simulink model "DroopControl"  (R2025b)
settings: Solver=VariableStepAuto  StartTime=0.0  StopTime=0.3  MaxStep=1/20e3/100  RelTol=1e-3
InitFcn:
  | fs = 20000;
  | Ts = 1/fs;
  | I2B = 10;
  | UB = 20;
  | freq0 = 50;
  | freqc = 0.29999999999999999;
  | w0 = 2*pi*freq0;
  | wc = 2*pi*freqc;
  | I2_Kp = 3.023;
  | I2_Kr = 16.36;
  | Uc_Kp = 0.010579843316015665;
  | Uc_Kr = 0.56544574743993026;
  | I1_Kpi = 1.73;
  | UDC = 48;
  | Ic_Kd = 0;
  | Ts2 = 1/500;
  | 
  | %% 20V / 12A droop-grid configuration
  | % wc_grid is separate from the existing QPR parameter wc.
  | Grid_Condition = 'STRONG'; % STRONG / WEAK_INDUCTIVE / WEAK_RESISTIVE
  | fn = 50;
  | wn = 2*pi*fn;
  | E0 = 20; % phase-voltage peak, V
  | I_base = 12; % current peak, A
  | S_inv = 1.5*E0*I_base;
  | Z_base = E0/I_base;
  | switch Grid_Condition
  |     case 'STRONG'
  |         SCR = 10;
  |         XR_ratio = 5;
  |         Sn = 10*S_inv;
  |         delta_f_max = 0.2;
  |         delta_E_max = 0.02*E0;
  |         grid_wc = 25; % power-filter cutoff, rad/s
  |     case 'WEAK_INDUCTIVE'
  |         SCR = 1.5;
  |         XR_ratio = 3;
  |         Sn = 1.5*S_inv;
  |         delta_f_max = 1.5;
  |         delta_E_max = 0.10*E0;
  |         grid_wc = 120;
  |     case 'WEAK_RESISTIVE'
  |         SCR = 1.5;
  |         XR_ratio = 1;
  |         Sn = 1.5*S_inv;
  |         delta_f_max = 1.5;
  |         delta_E_max = 0.10*E0;
  |         grid_wc = 120;
  |     otherwise
  |         error('DroopGrid:InvalidCondition','Unknown Grid_Condition: %s',Grid_Condition);
  | end
  | Z_grid = Z_base/SCR;
  | Rg_val = Z_grid/sqrt(1+XR_ratio^2);
  | Lg_val = Rg_val*XR_ratio/wn;
  | grid_mp = 2*pi*delta_f_max/Sn;
  | grid_nq = delta_E_max/Sn;
  | grid_p0 = 0;
  | grid_q0 = 0;
  | Ts_ctrl = 1e-4; % actual droop-grid update period, 10 kHz
  | 
  | %% Physical-unit voltage/current cascade parameters (2026-10-03)
  | LCL_L1 = 200e-6;
  | LCL_L2 = 47e-6;
  | LCL_C = 1.8e-05;
  | LCL_R1 = 0.029999999999999999;
  | LCL_R2 = 0.014999999999999999;
  | I_meas_base = 1; % Clarke output in A, without current normalization
  | U_meas_base = 1; % Clarke output in V, without voltage normalization
  | PWM_Vbase = 1; % SVPWM input in V; conversion gain is unity
  | % Original QPR code has resonant gain 2*Kr at its center frequency.
  | % Imported Kr is interpreted using 2*Kr*wc*s/(s^2+2*wc*s+w0^2).
  | Uc_Kr_Code = Uc_Kr/2;
  | % Analysis metadata only; these do not add a delay/Pade block.
  | Design_delay_s = 5.4999999999999995e-05;
  | Design_pade_order = 2;
  | 
  | % Imported conservative controller profile (2026-10-04)
  | % Source export: 2026-10-04T06:14:23.773Z
  | % QPR fixed center 50 Hz; controller input latch and presync follow selected experiment.
  | % Design_delay_s is analysis metadata, not an additional runtime delay.
  | % Inverter-side loads are Resistor1/4/5; grid-side loads unchanged.
model workspace (MAT data in the model file):
  CurrentTestFinalPeak = 0.3
  CurrentTestInitialPeak = 0.1
  CurrentTestSignedStepTime = 0.03
libraries: nesl_utility x31, fl_lib x28, ee_lib x27, simulink x1, eePowerMeasurement x1
(part 1 of 2)
settings Model: Creator=GoodUser  LastModifiedBy=GoodUser

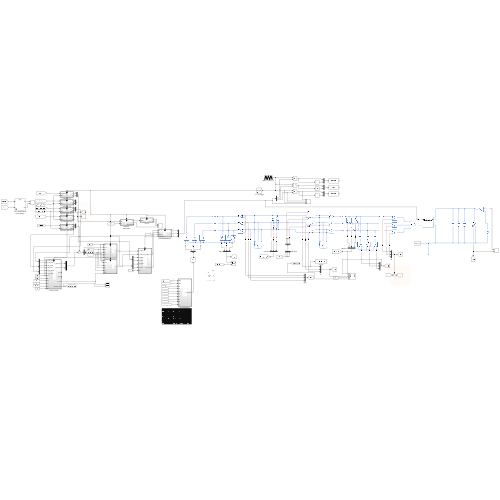
[thumbnail: Simulink's stored preview of the top-level diagram]
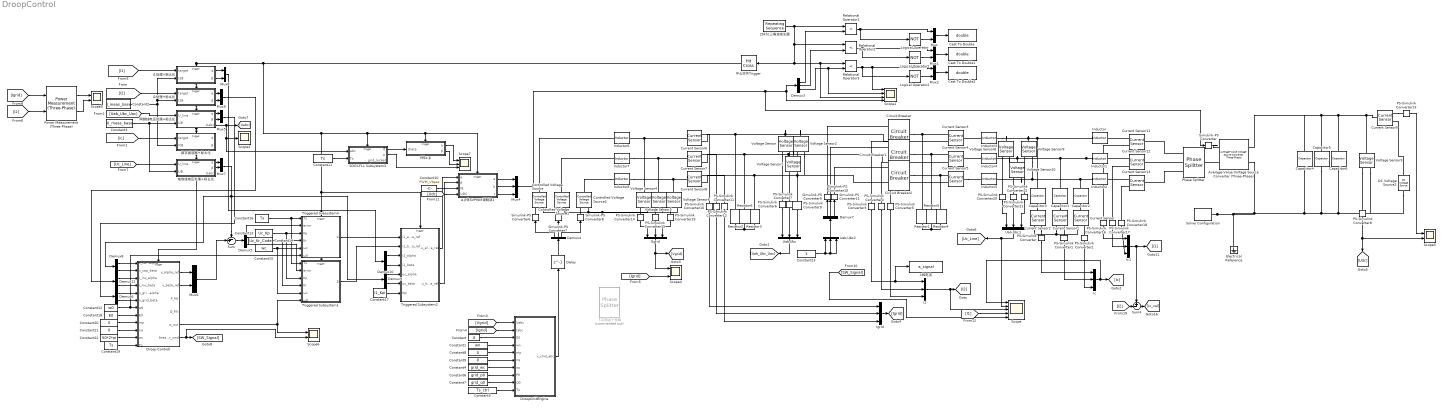
== system DroopControl ==
  20khz三角波发生器 : simulink/Sources/Repeating Sequence  rep_seq_t=[0 Ts/2 Ts]  rep_seq_y=[0 1 0]
  Average-Value Voltage Source Converter (Three-Phase) : ee_lib/Semiconductors & Converters/Converters/Average-Value Voltage Source Converter (Three-Phase)  port_option=ee.enum.threePhasePort.composite  frequency_option=ee.enum.converters.frequency.variable  input_option=ee.enum.converters.inputOption.ModWave  FRated=60 Hz  losses_parameterization=ee.enum.converters.losses.fixed  Pfixed=1 W  ks=0.01  kc1=1.7 V  kc2=0.01 Ohm  Ploss_vect=[100, 800, 1870, 3250, 4900] W  Irms_vect=[10, 100, 200, 300, 400] A  Vdc_nom=300 V  thermal_mass=30000 J/K  temperature_specify=off  temperature_priority=High  temperature=298.15 K  temperature_nominal_specify=off  temperature_nominal_value=1  temperature_nominal_unit=K
      settings: InternalSimscapePortConfiguration="{\"Bottom\":[],\"Left\":[{\"id\":\"ModWave\",\"label\":\"ModWave\",\"type\":\"input\"},{\"id\":\"N\",\"label\":\"~\",\"type\":\"foundation.electrical.three_phase\"}],\"Right\":[{\"id\":\"p\",\"label\":\"+\",\"type\":\"foundation.electrical.electrical\"},{\"id\":\"n\",\"label\":\"-\",\"type\":\"foundation.electrical.electrical\"}],\"Top\":[]}"
  A相电流 : ToWorkspace  VariableName=a_signal  SaveFormat=Timeseries  SampleTime=-1
  Capacitor1 : ee_lib/Passive/Capacitor  cap_option=ee.enum.passive.capacitor.capOption.const  c=LCL_C F  Cvec=[1e-05, 1e-06] F  Vvec=[0, 10] V  CV_table_symmetry=ee.enum.passive.capacitor.tableSymmetry.yes  f_vec=[1, 10] kHz  DFext_vec=[.8, 1.2]  enable_C_tol=ee.enum.toleranceApplication.none  averaging_period=0 s  C_tol=5  tol_distribution=ee.enum.toleranceDistribution.uniform  nSigma=4  r=8e-3 Ohm  g=0 1/Ohm  enable_operating_limits=ee.enum.enable.no  operating_limit_action=ee.enum.passive.reportOpLim.warn  max_working_voltage_range=[-25, 25] V  power_rating=1 W  maxTemperature=85 degC  thermalEnable=false  thermalMass=1 J/K  i_specify=off  i_priority=None  i=0 A  i_nominal_specify=off  i_nominal_value=1  i_nominal_unit=A  v_specify=off  v_priority=None  v=0 V  v_nominal_specify=off  v_nominal_value=1  v_nominal_unit=V  vc_specify=off  vc_priority=High  vc=0 V  vc_nominal_specify=off  vc_nominal_value=1  vc_nominal_unit=V  T_specify=off  T_priority=None  T=298.15 K  T_nominal_specify=off  T_nominal_value=1  T_nominal_unit=K
  Capacitor2 : ee_lib/Passive/Capacitor  cap_option=ee.enum.passive.capacitor.capOption.const  c=LCL_C F  Cvec=[1e-05, 1e-06] F  Vvec=[0, 10] V  CV_table_symmetry=ee.enum.passive.capacitor.tableSymmetry.yes  f_vec=[1, 10] kHz  DFext_vec=[.8, 1.2]  enable_C_tol=ee.enum.toleranceApplication.none  averaging_period=0 s  C_tol=5  tol_distribution=ee.enum.toleranceDistribution.uniform  nSigma=4  r=8e-3 Ohm  g=0 1/Ohm  enable_operating_limits=ee.enum.enable.no  operating_limit_action=ee.enum.passive.reportOpLim.warn  max_working_voltage_range=[-25, 25] V  power_rating=1 W  maxTemperature=85 degC  thermalEnable=false  thermalMass=1 J/K  i_specify=off  i_priority=None  i=0 A  i_nominal_specify=off  i_nominal_value=1  i_nominal_unit=A  v_specify=off  v_priority=None  v=0 V  v_nominal_specify=off  v_nominal_value=1  v_nominal_unit=V  vc_specify=off  vc_priority=High  vc=0 V  vc_nominal_specify=off  vc_nominal_value=1  vc_nominal_unit=V  T_specify=off  T_priority=None  T=298.15 K  T_nominal_specify=off  T_nominal_value=1  T_nominal_unit=K
  Capacitor3 : ee_lib/Passive/Capacitor  cap_option=ee.enum.passive.capacitor.capOption.const  c=LCL_C F  Cvec=[1e-05, 1e-06] F  Vvec=[0, 10] V  CV_table_symmetry=ee.enum.passive.capacitor.tableSymmetry.yes  f_vec=[1, 10] kHz  DFext_vec=[.8, 1.2]  enable_C_tol=ee.enum.toleranceApplication.none  averaging_period=0 s  C_tol=5  tol_distribution=ee.enum.toleranceDistribution.uniform  nSigma=4  r=8e-3 Ohm  g=0 1/Ohm  enable_operating_limits=ee.enum.enable.no  operating_limit_action=ee.enum.passive.reportOpLim.warn  max_working_voltage_range=[-25, 25] V  power_rating=1 W  maxTemperature=85 degC  thermalEnable=false  thermalMass=1 J/K  i_specify=off  i_priority=None  i=0 A  i_nominal_specify=off  i_nominal_value=1  i_nominal_unit=A  v_specify=off  v_priority=None  v=0 V  v_nominal_specify=off  v_nominal_value=1  v_nominal_unit=V  vc_specify=off  vc_priority=High  vc=0 V  vc_nominal_specify=off  vc_nominal_value=1  vc_nominal_unit=V  T_specify=off  T_priority=None  T=298.15 K  T_nominal_specify=off  T_nominal_value=1  T_nominal_unit=K
  Capacitor4 : ee_lib/Passive/Capacitor  cap_option=ee.enum.passive.capacitor.capOption.const  c=0.001 F  Cvec=[1e-05, 1e-06] F  Vvec=[0, 10] V  CV_table_symmetry=ee.enum.passive.capacitor.tableSymmetry.yes  f_vec=[1, 10] kHz  DFext_vec=[.8, 1.2]  enable_C_tol=ee.enum.toleranceApplication.none  averaging_period=0 s  C_tol=5  tol_distribution=ee.enum.toleranceDistribution.uniform  nSigma=4  r=200e-3 Ohm  g=0 1/Ohm  enable_operating_limits=ee.enum.enable.no  operating_limit_action=ee.enum.passive.reportOpLim.warn  max_working_voltage_range=[-25, 25] V  power_rating=1 W  maxTemperature=85 degC  thermalEnable=false  thermalMass=1 J/K  i_specify=off  i_priority=None  i=0 A  i_nominal_specify=off  i_nominal_value=1  i_nominal_unit=A  v_specify=on  v_priority=None  v=34.641 V  v_nominal_specify=off  v_nominal_value=1  v_nominal_unit=V  vc_specify=on  vc_priority=High  vc=34.641 V  vc_nominal_specify=off  vc_nominal_value=1  vc_nominal_unit=V  T_specify=off  T_priority=None  T=298.15 K  T_nominal_specify=off  T_nominal_value=1  T_nominal_unit=K
  Capacitor5 : ee_lib/Passive/Capacitor  cap_option=ee.enum.passive.capacitor.capOption.const  c=0.001 F  Cvec=[1e-05, 1e-06] F  Vvec=[0, 10] V  CV_table_symmetry=ee.enum.passive.capacitor.tableSymmetry.yes  f_vec=[1, 10] kHz  DFext_vec=[.8, 1.2]  enable_C_tol=ee.enum.toleranceApplication.none  averaging_period=0 s  C_tol=5  tol_distribution=ee.enum.toleranceDistribution.uniform  nSigma=4  r=200e-3 Ohm  g=0 1/Ohm  enable_operating_limits=ee.enum.enable.no  operating_limit_action=ee.enum.passive.reportOpLim.warn  max_working_voltage_range=[-25, 25] V  power_rating=1 W  maxTemperature=85 degC  thermalEnable=false  thermalMass=1 J/K  i_specify=off  i_priority=None  i=0 A  i_nominal_specify=off  i_nominal_value=1  i_nominal_unit=A  v_specify=on  v_priority=None  v=34.641 V  v_nominal_specify=off  v_nominal_value=1  v_nominal_unit=V  vc_specify=on  vc_priority=High  vc=34.641 V  vc_nominal_specify=off  vc_nominal_value=1  vc_nominal_unit=V  T_specify=off  T_priority=None  T=298.15 K  T_nominal_specify=off  T_nominal_value=1  T_nominal_unit=K
  Capacitor6 : ee_lib/Passive/Capacitor  cap_option=ee.enum.passive.capacitor.capOption.const  c=0.001 F  Cvec=[1e-05, 1e-06] F  Vvec=[0, 10] V  CV_table_symmetry=ee.enum.passive.capacitor.tableSymmetry.yes  f_vec=[1, 10] kHz  DFext_vec=[.8, 1.2]  enable_C_tol=ee.enum.toleranceApplication.none  averaging_period=0 s  C_tol=5  tol_distribution=ee.enum.toleranceDistribution.uniform  nSigma=4  r=200e-3 Ohm  g=0 1/Ohm  enable_operating_limits=ee.enum.enable.no  operating_limit_action=ee.enum.passive.reportOpLim.warn  max_working_voltage_range=[-25, 25] V  power_rating=1 W  maxTemperature=85 degC  thermalEnable=false  thermalMass=1 J/K  i_specify=off  i_priority=None  i=0 A  i_nominal_specify=off  i_nominal_value=1  i_nominal_unit=A  v_specify=on  v_priority=None  v=34.641 V  v_nominal_specify=off  v_nominal_value=1  v_nominal_unit=V  vc_specify=on  vc_priority=High  vc=34.641 V  vc_nominal_specify=off  vc_nominal_value=1  vc_nominal_unit=V  T_specify=off  T_priority=None  T=298.15 K  T_nominal_specify=off  T_nominal_value=1  T_nominal_unit=K
  Cast To Double : DataTypeConversion  OutDataTypeStr=double  SaturateOnIntegerOverflow=off  RndMeth=Floor
  Cast To Double1 : DataTypeConversion  OutDataTypeStr=double  SaturateOnIntegerOverflow=off  RndMeth=Floor
  Cast To Double2 : DataTypeConversion  OutDataTypeStr=double  SaturateOnIntegerOverflow=off  RndMeth=Floor
  Circuit Breaker : ee_lib/Switches & Breakers/Circuit Breaker  R_closed=0.001 Ohm  G_open=1e-6 1/Ohm  threshold=0.5 V  breaker_behavior=ee.enum.switches.breakerBehavior.zeroCrossingEnable
      settings: InternalSimscapePortConfiguration="{\"Bottom\":[],\"Left\":[{\"id\":\"vT\",\"label\":\"vT\",\"type\":\"input\"},{\"id\":\"p1\",\"label\":\"\",\"type\":\"foundation.electrical.electrical\"}],\"Right\":[{\"id\":\"p2\",\"label\":\"\",\"type\":\"foundation.electrical.electrical\"}],\"Top\":[]}"
  Circuit Breaker1 : ee_lib/Switches & Breakers/Circuit Breaker  R_closed=0.001 Ohm  G_open=1e-6 1/Ohm  threshold=0.5 V  breaker_behavior=ee.enum.switches.breakerBehavior.zeroCrossingEnable
      settings: InternalSimscapePortConfiguration="{\"Bottom\":[],\"Left\":[{\"id\":\"vT\",\"label\":\"vT\",\"type\":\"input\"},{\"id\":\"p1\",\"label\":\"\",\"type\":\"foundation.electrical.electrical\"}],\"Right\":[{\"id\":\"p2\",\"label\":\"\",\"type\":\"foundation.electrical.electrical\"}],\"Top\":[]}"
  Circuit Breaker2 : ee_lib/Switches & Breakers/Circuit Breaker  R_closed=0.001 Ohm  G_open=1e-6 1/Ohm  threshold=1 V  breaker_behavior=ee.enum.switches.breakerBehavior.zeroCrossingEnable
      settings: InternalSimscapePortConfiguration="{\"Bottom\":[],\"Left\":[{\"id\":\"vT\",\"label\":\"vT\",\"type\":\"input\"},{\"id\":\"p1\",\"label\":\"\",\"type\":\"foundation.electrical.electrical\"}],\"Right\":[{\"id\":\"p2\",\"label\":\"\",\"type\":\"foundation.electrical.electrical\"}],\"Top\":[]}"
  Constant{,8..9,20..21} (5 alike) : Constant  Value=0
  Constant1 : Constant  Value=wn
  Constant10 : Constant  Value=PWM_Vbase
  Constant11 : Constant  Value=Ts
  Constant12 : Constant  Value=w0
  Constant13 : Constant  Value=Uc_Kp
  Constant14 : Constant  Value=Uc_Kr_Code
  Constant15 : Constant  Value=wc
  Constant16 : Constant  Value=Ts
  Constant17 : Constant  Value=I1_Kpi
  Constant18 : Constant  Value=E0
  Constant19 : Constant  Value=Ts
  Constant2 : Constant  Value=I_meas_base
  Constant22 : Constant  Value=50*2*pi
  Constant23 : Constant
  Constant3 : Constant  Value=U_meas_base
  Constant4 : Constant  Value=grid_wc
  Constant5 : Constant  Value=Ts_ctrl
  Constant6 : Constant  Value=grid_p0
  Constant7 : Constant  Value=grid_q0
  Controlled Voltage Source : fl_lib/Electrical/Electrical Sources/Controlled Voltage Source
  Controlled Voltage Source1 : fl_lib/Electrical/Electrical Sources/Controlled Voltage Source
  Controlled Voltage Source2 : fl_lib/Electrical/Electrical Sources/Controlled Voltage Source
  Current Sensor{,1..9,11..13} (13 alike) : fl_lib/Electrical/Electrical Sensors/Current Sensor
  DC Voltage Source2 : fl_lib/Electrical/Electrical Sources/DC Voltage Source  v0=48 V
  Delay : Delay  DelayLength=1  InitialCondition=0
  Demux{5..6,8..11} (6 alike) : Demux  Outputs=2
  Demux3 : Demux  Outputs=3
  Demux4 : Demux  Outputs=3
  Demux7 : Demux  Outputs=3
  "Droop Controll " : Subsystem  TreatAsAtomicUnit=on
  DroopGridEngine : Subsystem  TreatAsAtomicUnit=on
  Electrical Reference : fl_lib/Electrical/Electrical Elements/Electrical Reference
  Ggrid : Mux  Inputs=3
  I1处理+标幺化 : Subsystem  TreatAsAtomicUnit=on
  I2 : Mux  Inputs=3
  I2处理+标幺化 : Subsystem  TreatAsAtomicUnit=on
  Ic : Mux  Inputs=3
  Ic1 : Mux  Inputs=3
  Igrid : Mux  Inputs=3
  Inductor : ee_lib/Passive/Inductor  l=LCL_L1 H  enable_L_tol=ee.enum.toleranceApplication.none  L_tol=20  tol_distribution=ee.enum.toleranceDistribution.uniform  nSigma=4  r=LCL_R1 Ohm  g=1e-9 1/Ohm  enable_operating_limits=ee.enum.enable.no  operating_limit_action=ee.enum.passive.reportOpLim.warn  max_working_current=1 A  power_rating=1 W  i_L_specify=off  i_L_priority=High  i_L=0 A  i_L_nominal_specify=off  i_L_nominal_value=1  i_L_nominal_unit=A
  Inductor1 : ee_lib/Passive/Inductor  l=LCL_L1 H  enable_L_tol=ee.enum.toleranceApplication.none  L_tol=20  tol_distribution=ee.enum.toleranceDistribution.uniform  nSigma=4  r=LCL_R1 Ohm  g=1e-9 1/Ohm  enable_operating_limits=ee.enum.enable.no  operating_limit_action=ee.enum.passive.reportOpLim.warn  max_working_current=1 A  power_rating=1 W  i_L_specify=off  i_L_priority=High  i_L=0 A  i_L_nominal_specify=off  i_L_nominal_value=1  i_L_nominal_unit=A
  Inductor2 : ee_lib/Passive/Inductor  l=LCL_L1 H  enable_L_tol=ee.enum.toleranceApplication.none  L_tol=20  tol_distribution=ee.enum.toleranceDistribution.uniform  nSigma=4  r=LCL_R1 Ohm  g=1e-9 1/Ohm  enable_operating_limits=ee.enum.enable.no  operating_limit_action=ee.enum.passive.reportOpLim.warn  max_working_current=1 A  power_rating=1 W  i_L_specify=off  i_L_priority=High  i_L=0 A  i_L_nominal_specify=off  i_L_nominal_value=1  i_L_nominal_unit=A
  Inductor3 : ee_lib/Passive/Inductor  l=LCL_L2 H  enable_L_tol=ee.enum.toleranceApplication.none  L_tol=20  tol_distribution=ee.enum.toleranceDistribution.uniform  nSigma=4  r=LCL_R2 Ohm  g=1e-9 1/Ohm  enable_operating_limits=ee.enum.enable.no  operating_limit_action=ee.enum.passive.reportOpLim.warn  max_working_current=1 A  power_rating=1 W  i_L_specify=off  i_L_priority=High  i_L=0 A  i_L_nominal_specify=off  i_L_nominal_value=1  i_L_nominal_unit=A
  Inductor4 : ee_lib/Passive/Inductor  l=LCL_L2 H  enable_L_tol=ee.enum.toleranceApplication.none  L_tol=20  tol_distribution=ee.enum.toleranceDistribution.uniform  nSigma=4  r=LCL_R2 Ohm  g=1e-9 1/Ohm  enable_operating_limits=ee.enum.enable.no  operating_limit_action=ee.enum.passive.reportOpLim.warn  max_working_current=1 A  power_rating=1 W  i_L_specify=off  i_L_priority=High  i_L=0 A  i_L_nominal_specify=off  i_L_nominal_value=1  i_L_nominal_unit=A
  Inductor5 : ee_lib/Passive/Inductor  l=LCL_L2 H  enable_L_tol=ee.enum.toleranceApplication.none  L_tol=20  tol_distribution=ee.enum.toleranceDistribution.uniform  nSigma=4  r=LCL_R2 Ohm  g=1e-9 1/Ohm  enable_operating_limits=ee.enum.enable.no  operating_limit_action=ee.enum.passive.reportOpLim.warn  max_working_current=1 A  power_rating=1 W  i_L_specify=off  i_L_priority=High  i_L=0 A  i_L_nominal_specify=off  i_L_nominal_value=1  i_L_nominal_unit=A
  Inductor6 : ee_lib/Passive/Inductor  l=Lg_val H  enable_L_tol=ee.enum.toleranceApplication.none  L_tol=20  tol_distribution=ee.enum.toleranceDistribution.uniform  nSigma=4  r=Rg_val Ohm  g=1e-9 1/Ohm  enable_operating_limits=ee.enum.enable.no  operating_limit_action=ee.enum.passive.reportOpLim.warn  max_working_current=1 A  power_rating=1 W  i_L_specify=off  i_L_priority=High  i_L=0 A  i_L_nominal_specify=off  i_L_nominal_value=1  i_L_nominal_unit=A
  Inductor7 : ee_lib/Passive/Inductor  l=Lg_val H  enable_L_tol=ee.enum.toleranceApplication.none  L_tol=20  tol_distribution=ee.enum.toleranceDistribution.uniform  nSigma=4  r=Rg_val Ohm  g=1e-9 1/Ohm  enable_operating_limits=ee.enum.enable.no  operating_limit_action=ee.enum.passive.reportOpLim.warn  max_working_current=1 A  power_rating=1 W  i_L_specify=off  i_L_priority=High  i_L=0 A  i_L_nominal_specify=off  i_L_nominal_value=1  i_L_nominal_unit=A
  Inductor8 : ee_lib/Passive/Inductor  l=Lg_val H  enable_L_tol=ee.enum.toleranceApplication.none  L_tol=20  tol_distribution=ee.enum.toleranceDistribution.uniform  nSigma=4  r=Rg_val Ohm  g=1e-9 1/Ohm  enable_operating_limits=ee.enum.enable.no  operating_limit_action=ee.enum.passive.reportOpLim.warn  max_working_current=1 A  power_rating=1 W  i_L_specify=off  i_L_priority=High  i_L=0 A  i_L_nominal_specify=off  i_L_nominal_value=1  i_L_nominal_unit=A
  Logical Operator : Logic  Operator=NOT  AllPortsSameDT=off  OutDataTypeStr=boolean
  Logical Operator1 : Logic  Operator=NOT  AllPortsSameDT=off  OutDataTypeStr=boolean
  Logical Operator2 : Logic  Operator=NOT  AllPortsSameDT=off  OutDataTypeStr=boolean
  Mux{,1..2,5..9} (8 alike) : Mux  Inputs=2
  Mux4 : Mux  Inputs=3
  PS-Simulink Converter{,1..22} (23 alike) : nesl_utility/PS-Simulink Converter  PhysicalDomain=network_engine_domain  SubClassName=ps_output  LeftPortType=input  RightPortType=output  PseudoPeriodic=off  Frequencies=[]  VectorFormat=inherit  Unit=inherit  AffineConversion=off
  Phase Splitter : ee_lib/Connectors & References/Phase Splitter
  Power Measurement (Three-Phase) : eePowerMeasurement/Power Measurement (Three-Phase)  LabelModeActiveChoice=Continuous  F=60  K=[0 1 2 3]  Seq=Positive  Ts=0
  Relational Operator1 : RelationalOperator  Operator=<  OutDataTypeStr=boolean  RndMeth=Simplest  InputSameDT=off
  Relational Operator2 : RelationalOperator  Operator=<  OutDataTypeStr=boolean  RndMeth=Simplest  InputSameDT=off
  Relational Operator3 : RelationalOperator  Operator=<  OutDataTypeStr=boolean  RndMeth=Simplest  InputSameDT=off
  Resistor1 : ee_lib/Passive/Resistor  R=50 Ohm  enable_R_tol=ee.enum.toleranceApplication.none  R_tol=5  tol_distribution=ee.enum.toleranceDistribution.uniform  nSigma=4  enable_operating_limits=ee.enum.enable.no  operating_limit_action=ee.enum.passive.reportOpLim.warn  power_rating=1 W  max_working_voltage=100 V  noise_mode=ee.enum.sources.noise.Disabled  Tdevice=25 degC  sample_time=1e-3 s  repeatability=ee.enum.ic.repeatability.notRepeatable  user_seed=0  auto_seed=3499211588  power_derating_T1=70 degC  power_derating_T2=155 degC  operating_temperature_range_vec=[-50, 150] degC  alpha=3.93e-3 1/K  Tmeas=25 degC  thermal_mass=100 J/K  temperature_specify=off  temperature_priority=High  temperature=298.15 K  temperature_nominal_specify=off  temperature_nominal_value=1  temperature_nominal_unit=K
  Resistor2 : ee_lib/Passive/Resistor  R=100 Ohm  enable_R_tol=ee.enum.toleranceApplication.none  R_tol=5  tol_distribution=ee.enum.toleranceDistribution.uniform  nSigma=4  enable_operating_limits=ee.enum.enable.no  operating_limit_action=ee.enum.passive.reportOpLim.warn  power_rating=1 W  max_working_voltage=100 V  noise_mode=ee.enum.sources.noise.Disabled  Tdevice=25 degC  sample_time=1e-3 s  repeatability=ee.enum.ic.repeatability.notRepeatable  user_seed=0  auto_seed=1826474873  power_derating_T1=70 degC  power_derating_T2=155 degC  operating_temperature_range_vec=[-50, 150] degC  alpha=3.93e-3 1/K  Tmeas=25 degC  thermal_mass=100 J/K  temperature_specify=off  temperature_priority=High  temperature=298.15 K  temperature_nominal_specify=off  temperature_nominal_value=1  temperature_nominal_unit=K
  Resistor3 : ee_lib/Passive/Resistor  R=100 Ohm  enable_R_tol=ee.enum.toleranceApplication.none  R_tol=5  tol_distribution=ee.enum.toleranceDistribution.uniform  nSigma=4  enable_operating_limits=ee.enum.enable.no  operating_limit_action=ee.enum.passive.reportOpLim.warn  power_rating=1 W  max_working_voltage=100 V  noise_mode=ee.enum.sources.noise.Disabled  Tdevice=25 degC  sample_time=1e-3 s  repeatability=ee.enum.ic.repeatability.notRepeatable  user_seed=0  auto_seed=693571696  power_derating_T1=70 degC  power_derating_T2=155 degC  operating_temperature_range_vec=[-50, 150] degC  alpha=3.93e-3 1/K  Tmeas=25 degC  thermal_mass=100 J/K  temperature_specify=off  temperature_priority=High  temperature=298.15 K  temperature_nominal_specify=off  temperature_nominal_value=1  temperature_nominal_unit=K
  Resistor4 : ee_lib/Passive/Resistor  R=50 Ohm  enable_R_tol=ee.enum.toleranceApplication.none  R_tol=5  tol_distribution=ee.enum.toleranceDistribution.uniform  nSigma=4  enable_operating_limits=ee.enum.enable.no  operating_limit_action=ee.enum.passive.reportOpLim.warn  power_rating=1 W  max_working_voltage=100 V  noise_mode=ee.enum.sources.noise.Disabled  Tdevice=25 degC  sample_time=1e-3 s  repeatability=ee.enum.ic.repeatability.notRepeatable  user_seed=0  auto_seed=3890346746  power_derating_T1=70 degC  power_derating_T2=155 degC  operating_temperature_range_vec=[-50, 150] degC  alpha=3.93e-3 1/K  Tmeas=25 degC  thermal_mass=100 J/K  temperature_specify=off  temperature_priority=High  temperature=298.15 K  temperature_nominal_specify=off  temperature_nominal_value=1  temperature_nominal_unit=K
  Resistor5 : ee_lib/Passive/Resistor  R=50 Ohm  enable_R_tol=ee.enum.toleranceApplication.none  R_tol=5  tol_distribution=ee.enum.toleranceDistribution.uniform  nSigma=4  enable_operating_limits=ee.enum.enable.no  operating_limit_action=ee.enum.passive.reportOpLim.warn  power_rating=1 W  max_working_voltage=100 V  noise_mode=ee.enum.sources.noise.Disabled  Tdevice=25 degC  sample_time=1e-3 s  repeatability=ee.enum.ic.repeatability.notRepeatable  user_seed=0  auto_seed=545404223  power_derating_T1=70 degC  power_derating_T2=155 degC  operating_temperature_range_vec=[-50, 150] degC  alpha=3.93e-3 1/K  Tmeas=25 degC  thermal_mass=100 J/K  temperature_specify=off  temperature_priority=High  temperature=298.15 K  temperature_nominal_specify=off  temperature_nominal_value=1  temperature_nominal_unit=K
  Resistor6 : ee_lib/Passive/Resistor  R=100 Ohm  enable_R_tol=ee.enum.toleranceApplication.none  R_tol=5  tol_distribution=ee.enum.toleranceDistribution.uniform  nSigma=4  enable_operating_limits=ee.enum.enable.no  operating_limit_action=ee.enum.passive.reportOpLim.warn  power_rating=1 W  max_working_voltage=100 V  noise_mode=ee.enum.sources.noise.Disabled  Tdevice=25 degC  sample_time=1e-3 s  repeatability=ee.enum.ic.repeatability.notRepeatable  user_seed=0  auto_seed=1343117392  power_derating_T1=70 degC  power_derating_T2=155 degC  operating_temperature_range_vec=[-50, 150] degC  alpha=3.93e-3 1/K  Tmeas=25 degC  thermal_mass=100 J/K  temperature_specify=off  temperature_priority=High  temperature=298.15 K  temperature_nominal_specify=off  temperature_nominal_value=1  temperature_nominal_unit=K
  SOGI-FLL Subsystem3 : Subsystem  TreatAsAtomicUnit=on
  Scope : Scope  NumInputPorts=5
      settings: ActiveDisplayYMinimum=-0.75702904285827766  ActiveDisplayYMaximum=0.7141001708324739
  Scope1 : Scope  NumInputPorts=4
      settings: ActiveDisplayYMinimum=-0.2219648833427319  ActiveDisplayYMaximum=1.3978468617731235
  Scope2 : Scope
      settings: ActiveDisplayYMinimum=-3.6838007228839231  ActiveDisplayYMaximum=2.775125553261212  DataLoggingVariableName=ScopeData2
  Scope{3..6} (4 alike) : Scope  NumInputPorts=2
      Scope3 settings: ActiveDisplayYMinimum=-5.9984838768546282  ActiveDisplayYMaximum=54.67249551752824  DataLoggingVariableName=ScopeData3
      Scope4 settings: ActiveDisplayYMinimum=-26.098635713677506  ActiveDisplayYMaximum=27.193712323408977  DataLoggingVariableName=ScopeData4
      Scope5 settings: ActiveDisplayYMinimum=-940.793349498487  ActiveDisplayYMaximum=150.37889545432691  DataLoggingVariableName=ScopeData5
      Scope6 settings: ActiveDisplayYMinimum=-39.269908169872409  ActiveDisplayYMaximum=353.42917352885172  DataLoggingVariableName=ScopeData6
  Scope7 : Scope  NumInputPorts=3
      settings: ActiveDisplayYMinimum=287.341337897508  ActiveDisplayYMaximum=314.82598204167613  DataLoggingVariableName=ScopeData7
  Simulink-PS Converter{,6..11} (7 alike) : nesl_utility/Simulink-PS Converter  PhysicalDomain=network_engine_domain  SubClassName=ps_input  LeftPortType=input  RightPortType=output  PseudoPeriodic=off  Frequencies=[]  NoiseDistribution=none  NoiseParameters=[]  Unit=1  AffineConversion=off  FilteringAndDerivatives=provide  SimscapeFilterOrder=1  InputFilterTimeConstant=0.001  UdotUserProvided=0
  Solver Configuration : nesl_utility/Solver Configuration  PhysicalDomain=network_engine_domain  SubClassName=solver  LeftPortType=input  RightPortType=generic  Tones=[]  Harmonics=[]  SimulateNoise=off  Profile=off  UseLocalSampling=off  EnableSwitchedLinearOptims=on  FrequencyDomain=off  UseCCode=off  RelTol=0.001  AbsTol=0.001  MinStep=1e-09  ToWorkspace=off  RevertToSquareIcSolve=off  NumHomotopyIterations=100  PhasorMode=off  PhasorModeNumHarmonics=1  ConsistencySolver=NEWTON_XTOL_AFTER_FTOL  IndexReductionMethod=DerivativeReplacement  DoDC=off  ResidualTolerance=1e-09  ConsistencyTolSource=GLOBAL  ConsistencyAbsTol=0.001  ConsistencyRelTol=0.001  ConsistencyTolFactor=0.001  UseLocalSolver=on  LocalSolverChoice=NE_BACKWARD_EULER_ADVANCER  ResolveIndetEquations=on  FunctionEvalNumThread=1  LocalSolverSampleTime=1/20e3/100  DoFixedCost=off  MaxNonlinIter=3  MaxModeIter=2  ComputeImpulses=off  ImpulseIterations=2  LinearAlgebra=auto  LinearAlgebraNumThread=0  EquationFormulation=NE_TIME_EF  DelaysMemoryBudget=1024  AutomaticFiltering=on  FilteringTimeConstant=0.001  PartitionStorageMethod=AS_NEEDED  PartitionMemoryBudget=1024  PartitionMethod=ROBUST  MultibodyUseLocalSolver=off  MultibodyLocalSolverChoice=ODE1  MultibodyLocalSolverSampleTime=0.001
  Sum : Sum  Inputs=-+|
  Sum4 : Sum  Inputs=+-|
  Triggered Subsystem1 : Subsystem  TreatAsAtomicUnit=on
  Triggered Subsystem2 : Subsystem  TreatAsAtomicUnit=on
  Triggered Subsystem4 : Subsystem  TreatAsAtomicUnit=on
  Uab,Ubc : Mux  Inputs=3
  Uab,Ubc1 : Mux  Inputs=3
  Uab,Ubc2 : Mux  Inputs=3
  Voltage Sensor{,1..6,8..10} (10 alike) : fl_lib/Electrical/Electrical Sensors/Voltage Sensor
  α,β转SVPWM调制波1 : Subsystem  TreatAsAtomicUnit=on
  θ转α,β : Subsystem  TreatAsAtomicUnit=on
  下次用这个布线 : ee_lib/Connectors & References/Phase Splitter  Commented=on
  中心对齐Trigger : HitCross  HitCrossingOffset=0.00  HitCrossingDirection=rising
  数字滤波器+标幺化 : Subsystem  TreatAsAtomicUnit=on
  电容线电压处理+标幺化 : Subsystem  TreatAsAtomicUnit=on
  网侧线电压处理+标幺化 : Subsystem  TreatAsAtomicUnit=on
  wires:
  PS-Simulink Converter/1 -> Ic/1
  PS-Simulink Converter1/1 -> Ic/2
  PS-Simulink Converter2/1 -> Ic/3
  PS-Simulink Converter3/1 -> A相电流/1, I2/1
  PS-Simulink Converter4/1 -> I2/2
  PS-Simulink Converter5/1 -> I2/3
  PS-Simulink Converter7/1 -> Uab,Ubc/2
  PS-Simulink Converter6/1 -> Uab,Ubc/1
  Demux3/1 -> Relational Operator1/2
  Relational Operator2/1 -> Mux1/1, Logical Operator1/1
  Demux3/2 -> Relational Operator2/2
  20khz三角波发生器/1 -> Relational Operator1/1, 中心对齐Trigger/1, Scope1/3, Relational Operator3/1, Relational Operator2/1
  Demux3/3 -> Scope1/2, Relational Operator3/2
  Mux/1 -> Cast To Double/1
  Mux1/1 -> Cast To Double1/1
  Ic/1 -> Scope/1, [Ic]
  Logical Operator1/1 -> Mux1/2
  Logical Operator/1 -> Mux/2
  Logical Operator2/1 -> Mux2/2
  Mux2/1 -> Cast To Double2/1
  Relational Operator3/1 -> Logical Operator2/1, Scope1/1, Mux2/1
  Relational Operator1/1 -> Logical Operator/1, Mux/1
  中心对齐Trigger/1 -> I1处理+标幺化/Trigger, 网侧线电压处理+标幺化/Trigger, "Droop Controll "/Trigger, 电容线电压处理+标幺化/Trigger, 数字滤波器+标幺化/Trigger, I2处理+标幺化/Trigger, SOGI-FLL Subsystem3/Trigger, α,β转SVPWM调制波1/Trigger, θ转α,β/Trigger, Triggered Subsystem2/Trigger, Triggered Subsystem1/Trigger, Triggered Subsystem4/Trigger
  I2/1 -> Scope/3, [I2]
  Uab,Ubc/1 -> [Uab_Ubc_Uac]
  [I2] -> I2处理+标幺化/1(target)
  [Uab_Ubc_Uac] -> 网侧线电压处理+标幺化/1(U_line)
  网侧线电压处理+标幺化/3(Uabc) -> Scope2/1, SOGI-FLL Subsystem3/1(abc), [Uabc]
  PS-Simulink Converter9/1 -> Uab,Ubc/3
  Constant2/1 -> 数字滤波器+标幺化/2(ICB), I1处理+标幺化/2(I2B), I2处理+标幺化/2(I2B)
  Constant3/1 -> 电容线电压处理+标幺化/2(UB), 网侧线电压处理+标幺化/2(UB)
  SOGI-FLL Subsystem3/1(θ) -> θ转α,β/1(theta)
  [Ic] -> 数字滤波器+标幺化/1(target)
  PS-Simulink Converter8/1 -> Scope3/2, [Udc]
  PS-Simulink Converter10/1 -> Igrid/1
  PS-Simulink Converter11/1 -> Igrid/2
  PS-Simulink Converter12/1 -> Igrid/3
  PS-Simulink Converter13/1 -> Scope3/1
  [I2] -> Power Measurement (Three-Phase)/2
  [Igrid] -> Power Measurement (Three-Phase)/1
  Power Measurement (Three-Phase)/1 -> Scope5/1
  Power Measurement (Three-Phase)/2 -> Scope5/2
  PS-Simulink Converter16/1 -> Ic1/1
  PS-Simulink Converter17/1 -> Ic1/2
  PS-Simulink Converter18/1 -> Ic1/3
  Ic1/1 -> [I1], Sum4/1
  [I2] -> Sum4/2
  Sum4/1 -> [Ic_cal]
  Igrid/1 -> [Igrid]
  [I1] -> I1处理+标幺化/1(target)
  DroopGridEngine/1(v_cmd_abc) -> Delay/1
  Demux4/1 -> Simulink-PS Converter6/1
  Demux4/2 -> Simulink-PS Converter7/1
  Demux4/3 -> Simulink-PS Converter8/1
  PS-Simulink Converter14/1 -> Ggrid/1
  PS-Simulink Converter15/1 -> Ggrid/2
  PS-Simulink Converter19/1 -> Ggrid/3
  Ggrid/1 -> [Vgrid], Scope4/1
  [Igrid] -> DroopGridEngine/2(Iabc)
  [Vgrid] -> DroopGridEngine/1(Vabc)
  Constant/1 -> DroopGridEngine/3(E0)
  Constant1/1 -> DroopGridEngine/4(wn)
  Constant4/1 -> DroopGridEngine/7(wc)
  Constant5/1 -> DroopGridEngine/10(Ts)
  Constant7/1 -> DroopGridEngine/9(Q0)
  Constant6/1 -> DroopGridEngine/8(P0)
  Constant9/1 -> DroopGridEngine/6(nq)
  Constant8/1 -> DroopGridEngine/5(mp)
  Mux4/1 -> Simulink-PS Converter/1, Demux3/1, Scope1/4
  Delay/1 -> Demux4/1
  [Igrid] -> Scope4/2
  "Droop Controll "/1(v_alpha_ref) -> Mux6/1
  "Droop Controll "/2(v_beta_ref) -> Mux6/2
  Mux6/1 -> Sum/2
  Sum/1 -> Demux5/1
  Demux5/1 -> Triggered Subsystem4/2(error)
  Demux5/2 -> Triggered Subsystem1/2(error)
  PS-Simulink Converter20/1 -> Uab,Ubc1/1
  PS-Simulink Converter21/1 -> Uab,Ubc1/2
  PS-Simulink Converter22/1 -> Uab,Ubc1/3
  Uab,Ubc1/1 -> Scope/2, [Uc_Line]
  [Uc_Line] -> 电容线电压处理+标幺化/1(U_line)
  Mux5/1 -> Demux6/1
  网侧线电压处理+标幺化/1(α) -> Mux5/1
  网侧线电压处理+标幺化/2(β) -> Mux5/2
  Constant11/1 -> SOGI-FLL Subsystem3/2(Ts)
  Demux7/1 -> Simulink-PS Converter9/1
  Demux7/2 -> Simulink-PS Converter10/1
  Demux7/3 -> Simulink-PS Converter11/1
  [SW_Signal] -> Scope/5
  Demux6/1 -> "Droop Controll "/5(v_grid_alpha)
  Demux6/2 -> "Droop Controll "/6(v_grid_beta)
  电容线电压处理+标幺化/1(α) -> Mux7/1
  电容线电压处理+标幺化/2(β) -> Mux7/2
  Demux8/1 -> "Droop Controll "/1(v_cap_alpha)
  Demux8/2 -> "Droop Controll "/2(v_cap_beta)
  Mux7/1 -> Demux9/1, Sum/1, Demux8/1
  Constant12/1 -> "Droop Controll "/7(w0), Triggered Subsystem4/6(ω0)
  Constant13/1 -> Triggered Subsystem4/3(Kp), Triggered Subsystem1/3(Kp)
  Constant14/1 -> Triggered Subsystem4/4(Kr), Triggered Subsystem1/4(Kr)
  Constant15/1 -> Triggered Subsystem4/5(ωc), Triggered Subsystem1/5(ωc)
  Constant16/1 -> Triggered Subsystem4/1(Ts), Triggered Subsystem1/1(Ts)
  Triggered Subsystem4/1(α) -> Triggered Subsystem2/1(i1_alpha_ref)
  Triggered Subsystem1/1(β) -> Triggered Subsystem2/2(i1_beta_ref)
  I1处理+标幺化/1(α) -> Mux8/1
  I1处理+标幺化/2(β) -> Mux8/2
  Mux8/1 -> Demux10/1
  Demux10/1 -> Triggered Subsystem2/3(i1_alpha)
  Demux10/2 -> Triggered Subsystem2/4(i1_beta)
  Demux9/1 -> Triggered Subsystem2/5(uc_alpha)
  Demux9/2 -> Triggered Subsystem2/6(uc_beta)
  Constant17/1 -> Triggered Subsystem2/7(Kpi)
  Triggered Subsystem2/1(u_alpha_ref) -> α,β转SVPWM调制波1/1(α)
  Triggered Subsystem2/2(u_beta_ref) -> α,β转SVPWM调制波1/2(β)
  α,β转SVPWM调制波1/1(a) -> Mux4/1
  α,β转SVPWM调制波1/2(b) -> Mux4/2
  α,β转SVPWM调制波1/3(c) -> Mux4/3
  Constant10/1 -> α,β转SVPWM调制波1/3(IB)
  [Udc] -> α,β转SVPWM调制波1/4(UDC)
  Constant18/1 -> "Droop Controll "/8(E0)
  Constant19/1 -> "Droop Controll "/12(Ts)
  Constant21/1 -> "Droop Controll "/10(nq)
  Constant20/1 -> "Droop Controll "/9(mp)
  Constant22/1 -> "Droop Controll "/11(wc)
  I2处理+标幺化/1(α) -> Mux9/1
  I2处理+标幺化/2(β) -> Mux9/2
  Mux9/1 -> Demux11/1
  Demux11/1 -> "Droop Controll "/3(i_inv_alpha)
  Demux11/2 -> "Droop Controll "/4(i_inv_beta)
  Constant23/1 -> Uab,Ubc2/2, Uab,Ubc2/3, Uab,Ubc2/1
  Uab,Ubc2/1 -> Demux7/1
  [I1] -> Scope/4
  "Droop Controll "/5(w_out) -> Scope6/1, Triggered Subsystem1/6(ω0)
  "Droop Controll "/6(breaker_cmd) -> Scope6/2, [SW_Signal]
  SOGI-FLL Subsystem3/2(ω) -> Scope7/3
  θ转α,β/1(α) -> Scope7/1
  θ转α,β/2(β) -> Scope7/2
  connections:
  Inductor/LConn1 -- Voltage Sensor9/LConn1 -- Voltage Sensor8/LConn1 -- Inductor3/RConn1 -- Capacitor3/LConn1
  Inductor1/LConn1 -- Inductor4/RConn1 -- Voltage Sensor8/RConn2 -- Voltage Sensor10/LConn1 -- Capacitor1/LConn1
  Capacitor2/LConn1 -- Voltage Sensor10/RConn2 -- Inductor5/RConn1 -- Voltage Sensor9/RConn2 -- Inductor2/LConn1
  Current Sensor1/RConn2 -- Current Sensor/RConn2 -- Current Sensor2/RConn2
  Inductor3/LConn1 -- Current Sensor3/LConn1
  Current Sensor/LConn1 -- Capacitor2/RConn1
  Capacitor1/RConn1 -- Current Sensor1/LConn1
  Capacitor3/RConn1 -- Current Sensor2/LConn1
  Current Sensor2/RConn1 -- PS-Simulink Converter/LConn1
  PS-Simulink Converter1/LConn1 -- Current Sensor1/RConn1
  PS-Simulink Converter2/LConn1 -- Current Sensor/RConn1
  Inductor4/LConn1 -- Current Sensor4/LConn1
  Current Sensor5/LConn1 -- Inductor5/LConn1
  Resistor6/LConn1 -- Voltage Sensor1/LConn1 -- Circuit Breaker1/LConn2 -- Voltage Sensor/RConn2 -- Current Sensor7/RConn2
  PS-Simulink Converter3/LConn1 -- Current Sensor3/RConn1
  Current Sensor4/RConn1 -- PS-Simulink Converter4/LConn1
  PS-Simulink Converter5/LConn1 -- Current Sensor5/RConn1
  Resistor2/LConn1 -- Circuit Breaker/LConn2 -- Voltage Sensor2/LConn1 -- Voltage Sensor/LConn1 -- Current Sensor6/RConn2
  Resistor3/LConn1 -- Circuit Breaker2/LConn2 -- Voltage Sensor2/RConn2 -- Voltage Sensor1/RConn2 -- Current Sensor8/RConn2
  Voltage Sensor3/RConn1 -- PS-Simulink Converter8/LConn1
  Current Sensor6/LConn1 -- Voltage Sensor4/LConn1 -- Inductor6/RConn1
  Current Sensor6/RConn1 -- PS-Simulink Converter10/LConn1
  Current Sensor7/RConn1 -- PS-Simulink Converter11/LConn1
  Current Sensor8/RConn1 -- PS-Simulink Converter12/LConn1
  Resistor3/RConn1 -- Resistor2/RConn1 -- Resistor6/RConn1
  Inductor7/RConn1 -- Voltage Sensor5/LConn1 -- Current Sensor7/LConn1
  Inductor8/RConn1 -- Voltage Sensor6/LConn1 -- Current Sensor8/LConn1
  Current Sensor9/RConn1 -- PS-Simulink Converter13/LConn1
  Voltage Sensor3/LConn1 -- Capacitor6/LConn1 -- Capacitor4/LConn1 -- Average-Value Voltage Source Converter (Three-Phase)/RConn1 -- Capacitor5/LConn1 -- Current Sensor9/LConn1
  Solver Configuration/RConn1 -- DC Voltage Source2/RConn1 -- Voltage Sensor3/RConn2 -- Capacitor6/RConn1 -- Capacitor5/RConn1 -- Capacitor4/RConn1 -- Average-Value Voltage Source Converter (Three-Phase)/RConn2 -- Electrical Reference/LConn1
  DC Voltage Source2/LConn1 -- Current Sensor9/RConn2
  Current Sensor11/RConn2 -- Inductor/RConn1
  Current Sensor12/RConn2 -- Inductor1/RConn1
  Inductor2/RConn1 -- Current Sensor13/RConn2
  Current Sensor11/RConn1 -- PS-Simulink Converter16/LConn1
  Current Sensor12/RConn1 -- PS-Simulink Converter17/LConn1
  Current Sensor13/RConn1 -- PS-Simulink Converter18/LConn1
  Controlled Voltage Source/LConn1 -- Inductor6/LConn1
  Inductor7/LConn1 -- Controlled Voltage Source1/LConn1
  Inductor8/LConn1 -- Controlled Voltage Source2/LConn1
  Simulink-PS Converter6/RConn1 -- Controlled Voltage Source/RConn1
  Simulink-PS Converter8/RConn1 -- Controlled Voltage Source2/RConn1
  Simulink-PS Converter7/RConn1 -- Controlled Voltage Source1/RConn1
  Controlled Voltage Source/RConn2 -- Voltage Sensor4/RConn2 -- Voltage Sensor6/RConn2 -- Voltage Sensor5/RConn2 -- Controlled Voltage Source2/RConn2 -- Controlled Voltage Source1/RConn2
  Voltage Sensor4/RConn1 -- PS-Simulink Converter14/LConn1
  PS-Simulink Converter15/LConn1 -- Voltage Sensor5/RConn1
  Voltage Sensor6/RConn1 -- PS-Simulink Converter19/LConn1
  PS-Simulink Converter20/LConn1 -- Voltage Sensor8/RConn1
  PS-Simulink Converter21/LConn1 -- Voltage Sensor10/RConn1
  Voltage Sensor9/RConn1 -- PS-Simulink Converter22/LConn1
  Simulink-PS Converter9/RConn1 -- Circuit Breaker/LConn1
  Simulink-PS Converter10/RConn1 -- Circuit Breaker1/LConn1
  Simulink-PS Converter11/RConn1 -- Circuit Breaker2/LConn1
  Circuit Breaker/RConn1 -- Resistor1/LConn1 -- Current Sensor3/RConn2
  Circuit Breaker1/RConn1 -- Resistor5/LConn1 -- Current Sensor4/RConn2
  Circuit Breaker2/RConn1 -- Resistor4/LConn1 -- Current Sensor5/RConn2
  Voltage Sensor/RConn1 -- PS-Simulink Converter6/LConn1
  Voltage Sensor1/RConn1 -- PS-Simulink Converter7/LConn1
  Voltage Sensor2/RConn1 -- PS-Simulink Converter9/LConn1
  Resistor4/RConn1 -- Resistor5/RConn1 -- Resistor1/RConn1
  Phase Splitter/RConn1 -- Current Sensor11/LConn1
  Phase Splitter/RConn2 -- Current Sensor12/LConn1
  Phase Splitter/RConn3 -- Current Sensor13/LConn1
  Average-Value Voltage Source Converter (Three-Phase)/LConn2 -- Phase Splitter/LConn1
  Simulink-PS Converter/RConn1 -- Average-Value Voltage Source Converter (Three-Phase)/LConn1

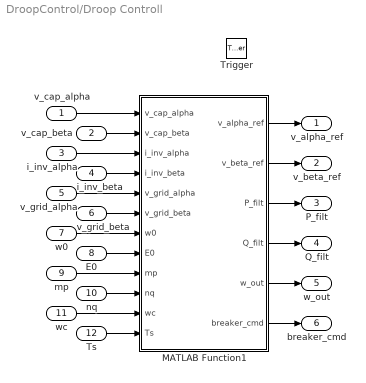
== system DroopControl/Droop Controll  ==
  v_cap_alpha : Inport
  v_cap_beta : Inport  Port=2
  i_inv_alpha : Inport  Port=3
  i_inv_beta : Inport  Port=4
  v_grid_alpha : Inport  Port=5
  v_grid_beta : Inport  Port=6
  w0 : Inport  Port=7
  E0 : Inport  Port=8
  mp : Inport  Port=9
  nq : Inport  Port=10
  wc : Inport  Port=11
  Ts : Inport  Port=12
  Trigger : TriggerPort  VariantControl=(inherit)
  MATLAB Function1 : MATLAB Function  TreatAsAtomicUnit=on
  v_alpha_ref : Outport
  v_beta_ref : Outport  Port=2
  P_filt : Outport  Port=3
  Q_filt : Outport  Port=4
  w_out : Outport  Port=5
  breaker_cmd : Outport  Port=6
  wires:
  Ts/1 -> MATLAB Function1/12(Ts)
  wc/1 -> MATLAB Function1/11(wc)
  nq/1 -> MATLAB Function1/10(nq)
  mp/1 -> MATLAB Function1/9(mp)
  E0/1 -> MATLAB Function1/8(E0)
  w0/1 -> MATLAB Function1/7(w0)
  MATLAB Function1/1(v_alpha_ref) -> v_alpha_ref/1
  MATLAB Function1/2(v_beta_ref) -> v_beta_ref/1
  MATLAB Function1/3(P_filt) -> P_filt/1
  MATLAB Function1/4(Q_filt) -> Q_filt/1
  MATLAB Function1/5(w_out) -> w_out/1
  v_grid_beta/1 -> MATLAB Function1/6(v_grid_beta)
  v_cap_alpha/1 -> MATLAB Function1/1(v_cap_alpha)
  v_cap_beta/1 -> MATLAB Function1/2(v_cap_beta)
  i_inv_alpha/1 -> MATLAB Function1/3(i_inv_alpha)
  i_inv_beta/1 -> MATLAB Function1/4(i_inv_beta)
  v_grid_alpha/1 -> MATLAB Function1/5(v_grid_alpha)
  MATLAB Function1/6(breaker_cmd) -> breaker_cmd/1

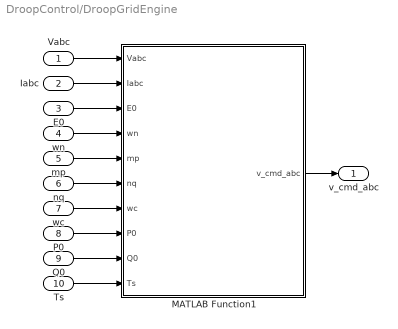
== system DroopControl/DroopGridEngine ==
  Vabc : Inport
  Iabc : Inport  Port=2
  E0 : Inport  Port=3
  wn : Inport  Port=4
  mp : Inport  Port=5
  nq : Inport  Port=6
  wc : Inport  Port=7
  P0 : Inport  Port=8
  Q0 : Inport  Port=9
  Ts : Inport  Port=10
  MATLAB Function1 : MATLAB Function  TreatAsAtomicUnit=on
  v_cmd_abc : Outport
  wires:
  MATLAB Function1/1(v_cmd_abc) -> v_cmd_abc/1
  Vabc/1 -> MATLAB Function1/1(Vabc)
  Iabc/1 -> MATLAB Function1/2(Iabc)
  Ts/1 -> MATLAB Function1/10(Ts)
  Q0/1 -> MATLAB Function1/9(Q0)
  P0/1 -> MATLAB Function1/8(P0)
  wc/1 -> MATLAB Function1/7(wc)
  nq/1 -> MATLAB Function1/6(nq)
  mp/1 -> MATLAB Function1/5(mp)
  wn/1 -> MATLAB Function1/4(wn)
  E0/1 -> MATLAB Function1/3(E0)

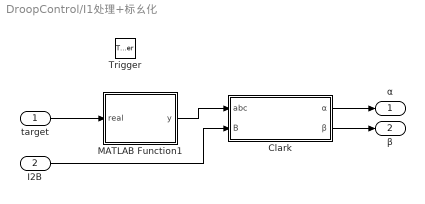
== system DroopControl/I1处理+标幺化 ==
  target : Inport  LatchByDelayingOutsideSignal=on
  I2B : Inport  Port=2
  Trigger : TriggerPort  VariantControl=(inherit)
  Clark : Subsystem  TreatAsAtomicUnit=on
  MATLAB Function1 : MATLAB Function  TreatAsAtomicUnit=on
  α : Outport
  β : Outport  Port=2
  wires:
  I2B/1 -> Clark/2(B)
  Clark/2(β) -> β/1
  Clark/1(α) -> α/1
  MATLAB Function1/1(y) -> Clark/1(abc)
  target/1 -> MATLAB Function1/1(real)

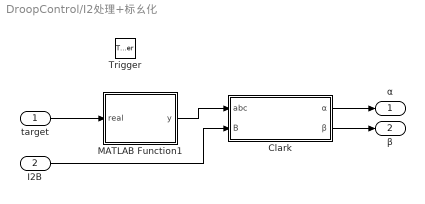
== system DroopControl/I2处理+标幺化 ==
  target : Inport  LatchByDelayingOutsideSignal=on
  I2B : Inport  Port=2
  Trigger : TriggerPort  VariantControl=(inherit)
  Clark : Subsystem  TreatAsAtomicUnit=on
  MATLAB Function1 : MATLAB Function  TreatAsAtomicUnit=on
  α : Outport
  β : Outport  Port=2
  wires:
  target/1 -> MATLAB Function1/1(real)
  MATLAB Function1/1(y) -> Clark/1(abc)
  Clark/1(α) -> α/1
  Clark/2(β) -> β/1
  I2B/1 -> Clark/2(B)

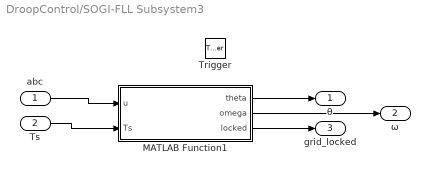
== system DroopControl/SOGI-FLL Subsystem3 ==
  abc : Inport
  Ts : Inport  Port=2
  Trigger : TriggerPort  VariantControl=(inherit)
  MATLAB Function1 : MATLAB Function  TreatAsAtomicUnit=on
  θ : Outport
  ω : Outport  Port=2
  grid_locked : Outport  Port=3
  wires:
  MATLAB Function1/2(omega) -> ω/1
  abc/1 -> MATLAB Function1/1(u)
  MATLAB Function1/1(theta) -> θ/1
  Ts/1 -> MATLAB Function1/2(Ts)
  MATLAB Function1/3(locked) -> grid_locked/1

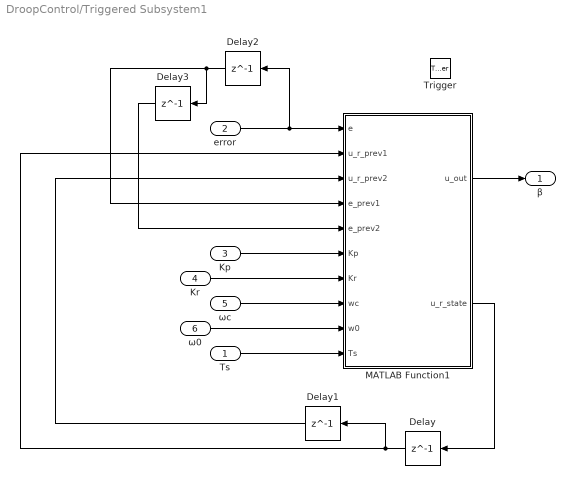
== system DroopControl/Triggered Subsystem1 ==
  Ts : Inport
  error : Inport  Port=2
  Kp : Inport  Port=3
  Kr : Inport  Port=4
  ωc : Inport  Port=5
  ω0 : Inport  Port=6
  Trigger : TriggerPort  VariantControl=(inherit)
  Delay{,1..3} (4 alike) : Delay  DelayLength=1  InitialCondition=0
  MATLAB Function1 : MATLAB Function  TreatAsAtomicUnit=on
  β : Outport
  wires:
  Delay3/1 -> MATLAB Function1/5(e_prev2)
  Delay2/1 -> MATLAB Function1/4(e_prev1), Delay3/1
  error/1 -> MATLAB Function1/1(e), Delay2/1
  Delay1/1 -> MATLAB Function1/3(u_r_prev2)
  Delay/1 -> MATLAB Function1/2(u_r_prev1), Delay1/1
  MATLAB Function1/2(u_r_state) -> Delay/1
  Kp/1 -> MATLAB Function1/6(Kp)
  Kr/1 -> MATLAB Function1/7(Kr)
  ωc/1 -> MATLAB Function1/8(wc)
  ω0/1 -> MATLAB Function1/9(w0)
  Ts/1 -> MATLAB Function1/10(Ts)
  MATLAB Function1/1(u_out) -> β/1

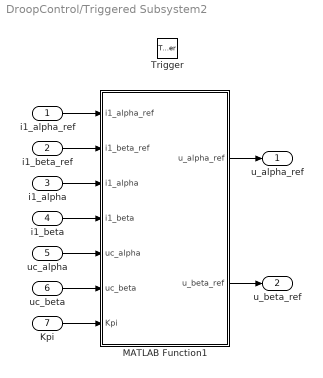
== system DroopControl/Triggered Subsystem2 ==
  i1_alpha_ref : Inport
  i1_beta_ref : Inport  Port=2
  i1_alpha : Inport  Port=3
  i1_beta : Inport  Port=4
  uc_alpha : Inport  Port=5
  uc_beta : Inport  Port=6
  Kpi : Inport  Port=7
  Trigger : TriggerPort  VariantControl=(inherit)
  MATLAB Function1 : MATLAB Function  TreatAsAtomicUnit=on
  u_alpha_ref : Outport
  u_beta_ref : Outport  Port=2
  wires:
  i1_alpha_ref/1 -> MATLAB Function1/1(i1_alpha_ref)
  Kpi/1 -> MATLAB Function1/7(Kpi)
  uc_beta/1 -> MATLAB Function1/6(uc_beta)
  uc_alpha/1 -> MATLAB Function1/5(uc_alpha)
  i1_beta/1 -> MATLAB Function1/4(i1_beta)
  i1_alpha/1 -> MATLAB Function1/3(i1_alpha)
  i1_beta_ref/1 -> MATLAB Function1/2(i1_beta_ref)
  MATLAB Function1/1(u_alpha_ref) -> u_alpha_ref/1
  MATLAB Function1/2(u_beta_ref) -> u_beta_ref/1

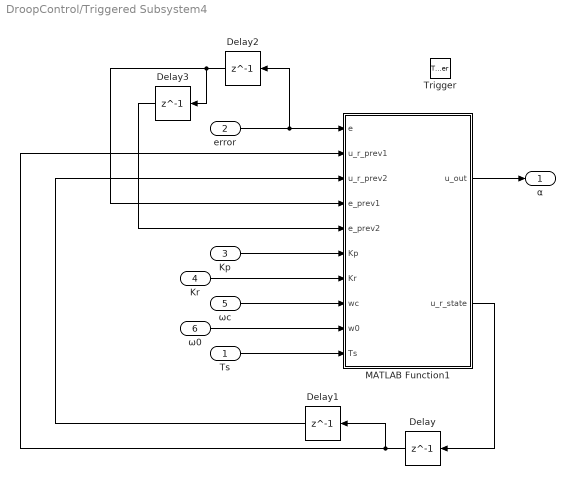
== system DroopControl/Triggered Subsystem4 ==
  Ts : Inport
  error : Inport  Port=2
  Kp : Inport  Port=3
  Kr : Inport  Port=4
  ωc : Inport  Port=5
  ω0 : Inport  Port=6
  Trigger : TriggerPort  VariantControl=(inherit)
  Delay{,1..3} (4 alike) : Delay  DelayLength=1  InitialCondition=0
  MATLAB Function1 : MATLAB Function  TreatAsAtomicUnit=on
  α : Outport
  wires:
  MATLAB Function1/1(u_out) -> α/1
  Ts/1 -> MATLAB Function1/10(Ts)
  ω0/1 -> MATLAB Function1/9(w0)
  ωc/1 -> MATLAB Function1/8(wc)
  Kr/1 -> MATLAB Function1/7(Kr)
  Kp/1 -> MATLAB Function1/6(Kp)
  MATLAB Function1/2(u_r_state) -> Delay/1
  Delay/1 -> Delay1/1, MATLAB Function1/2(u_r_prev1)
  Delay1/1 -> MATLAB Function1/3(u_r_prev2)
  error/1 -> Delay2/1, MATLAB Function1/1(e)
  Delay2/1 -> Delay3/1, MATLAB Function1/4(e_prev1)
  Delay3/1 -> MATLAB Function1/5(e_prev2)

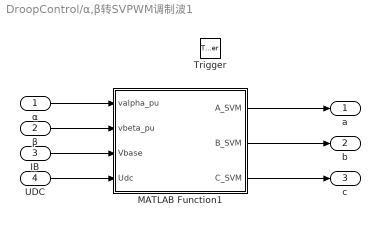
== system DroopControl/α,β转SVPWM调制波1 ==
  α : Inport
  β : Inport  Port=2
  IB : Inport  Port=3  LatchByDelayingOutsideSignal=on
  UDC : Inport  Port=4  LatchByDelayingOutsideSignal=on
  Trigger : TriggerPort  VariantControl=(inherit)
  MATLAB Function1 : MATLAB Function  TreatAsAtomicUnit=on
  a : Outport
  b : Outport  Port=2
  c : Outport  Port=3
  wires:
  MATLAB Function1/2(B_SVM) -> b/1
  α/1 -> MATLAB Function1/1(valpha_pu)
  MATLAB Function1/1(A_SVM) -> a/1
  MATLAB Function1/3(C_SVM) -> c/1
  β/1 -> MATLAB Function1/2(vbeta_pu)
  IB/1 -> MATLAB Function1/3(Vbase)
  UDC/1 -> MATLAB Function1/4(Udc)

== system DroopControl/θ转α,β ==
  theta : Inport
  Trigger : TriggerPort  VariantControl=(inherit)
  MATLAB Function1 : MATLAB Function  TreatAsAtomicUnit=on
  α : Outport
  β : Outport  Port=2
  wires:
  MATLAB Function1/1(alpha) -> α/1
  theta/1 -> MATLAB Function1/1(theta)
  MATLAB Function1/2(beta) -> β/1

== system DroopControl/数字滤波器+标幺化 ==
  target : Inport  LatchByDelayingOutsideSignal=on
  ICB : Inport  Port=2
  Trigger : TriggerPort  VariantControl=(inherit)
  Clark1 : Subsystem  TreatAsAtomicUnit=on
      settings: PortSchema="{\"entries\":[{\"content\":{\"sides\":[{\"content\":{\"connectorIds\":[\"In1\",\"In2\"]},\"type\":\"ConnectorPlacement.EquallySpacedRectSide\",\"uuid\":\"5266b147-56b7-4e2a-a13b-4b3ad7884dce\"},{\"content\":{\"connectorIds\":[\"Out1\",\"Out2\"],\"side\":\"RIGHT\"},\"type\":\"ConnectorPlacement.EquallySpacedRectSide\",\"uuid\":\"f7aac5c9-4e6b-4b0b-a99e-124a22eab803\"},{\"content\":{\"side\":\"TOP\"},\"type\":\"ConnectorPlacement.EquallySpacedRectSide\",\"uuid\":\"791bb2d5-f4db-46e5-b405-e7e666275d8b\"},{\"content\":{\"connectorIds\":[\"Out3\"],\"side\":\"BOTTOM\"},\"type\":\"ConnectorPlacement.EquallySpacedRectSide\",\"uuid\":\"b0b7b589-8650-446a-b530-e4865644ee8e\"}]},\"type\":\"ConnectorPlacement.EquallySpacedConnector\",\"uuid\":\"fa79ae73-0718-4a11-9c0b-03878e9e1adb\"}],\"packageUris\":[\"http://schema.mathworks.com/mf0/Connector/R2020b\"],\"version\":\"1.0\"}"
  MATLAB Function1 : MATLAB Function  TreatAsAtomicUnit=on
  α : Outport
  β : Outport  Port=2
  wires:
  target/1 -> MATLAB Function1/1(real)
  MATLAB Function1/1(y) -> Clark1/1(abc)
  Clark1/2(β) -> β/1
  Clark1/1(α) -> α/1
  ICB/1 -> Clark1/2(B)

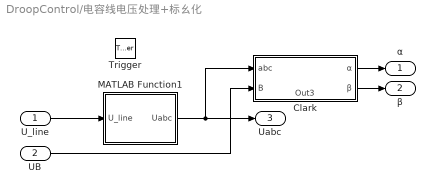
== system DroopControl/电容线电压处理+标幺化 ==
  U_line : Inport  LatchByDelayingOutsideSignal=on
  UB : Inport  Port=2
  Trigger : TriggerPort  VariantControl=(inherit)
  Clark : Subsystem  TreatAsAtomicUnit=on
      settings: PortSchema="{\"entries\":[{\"content\":{\"sides\":[{\"content\":{\"connectorIds\":[\"In1\",\"In2\"]},\"type\":\"ConnectorPlacement.EquallySpacedRectSide\",\"uuid\":\"5266b147-56b7-4e2a-a13b-4b3ad7884dce\"},{\"content\":{\"connectorIds\":[\"Out1\",\"Out2\"],\"side\":\"RIGHT\"},\"type\":\"ConnectorPlacement.EquallySpacedRectSide\",\"uuid\":\"f7aac5c9-4e6b-4b0b-a99e-124a22eab803\"},{\"content\":{\"side\":\"TOP\"},\"type\":\"ConnectorPlacement.EquallySpacedRectSide\",\"uuid\":\"791bb2d5-f4db-46e5-b405-e7e666275d8b\"},{\"content\":{\"connectorIds\":[\"Out3\"],\"side\":\"BOTTOM\"},\"type\":\"ConnectorPlacement.EquallySpacedRectSide\",\"uuid\":\"b0b7b589-8650-446a-b530-e4865644ee8e\"}]},\"type\":\"ConnectorPlacement.EquallySpacedConnector\",\"uuid\":\"fa79ae73-0718-4a11-9c0b-03878e9e1adb\"}],\"packageUris\":[\"http://schema.mathworks.com/mf0/Connector/R2020b\"],\"version\":\"1.0\"}"
  MATLAB Function1 : MATLAB Function  TreatAsAtomicUnit=on
  α : Outport
  β : Outport  Port=2
  Uabc : Outport  Port=3
  wires:
  UB/1 -> Clark/2(B)
  Clark/2(β) -> β/1
  Clark/1(α) -> α/1
  MATLAB Function1/1(Uabc) -> Uabc/1, Clark/1(abc)
  U_line/1 -> MATLAB Function1/1(U_line)

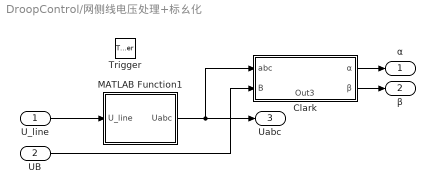
== system DroopControl/网侧线电压处理+标幺化 ==
  U_line : Inport  LatchByDelayingOutsideSignal=on
  UB : Inport  Port=2
  Trigger : TriggerPort  VariantControl=(inherit)
  Clark : Subsystem  TreatAsAtomicUnit=on
      settings: PortSchema="{\"entries\":[{\"content\":{\"sides\":[{\"content\":{\"connectorIds\":[\"In1\",\"In2\"]},\"type\":\"ConnectorPlacement.EquallySpacedRectSide\",\"uuid\":\"5266b147-56b7-4e2a-a13b-4b3ad7884dce\"},{\"content\":{\"connectorIds\":[\"Out1\",\"Out2\"],\"side\":\"RIGHT\"},\"type\":\"ConnectorPlacement.EquallySpacedRectSide\",\"uuid\":\"f7aac5c9-4e6b-4b0b-a99e-124a22eab803\"},{\"content\":{\"side\":\"TOP\"},\"type\":\"ConnectorPlacement.EquallySpacedRectSide\",\"uuid\":\"791bb2d5-f4db-46e5-b405-e7e666275d8b\"},{\"content\":{\"connectorIds\":[\"Out3\"],\"side\":\"BOTTOM\"},\"type\":\"ConnectorPlacement.EquallySpacedRectSide\",\"uuid\":\"b0b7b589-8650-446a-b530-e4865644ee8e\"}]},\"type\":\"ConnectorPlacement.EquallySpacedConnector\",\"uuid\":\"fa79ae73-0718-4a11-9c0b-03878e9e1adb\"}],\"packageUris\":[\"http://schema.mathworks.com/mf0/Connector/R2020b\"],\"version\":\"1.0\"}"
  MATLAB Function1 : MATLAB Function  TreatAsAtomicUnit=on
  α : Outport
  β : Outport  Port=2
  Uabc : Outport  Port=3
  wires:
  U_line/1 -> MATLAB Function1/1(U_line)
  MATLAB Function1/1(Uabc) -> Clark/1(abc), Uabc/1
  Clark/1(α) -> α/1
  Clark/2(β) -> β/1
  UB/1 -> Clark/2(B)

== system DroopControl/I1处理+标幺化/Clark ==
  abc : Inport
  B : Inport  Port=2
  MATLAB Function1 : MATLAB Function  TreatAsAtomicUnit=on
  α : Outport
  β : Outport  Port=2
  wires:
  B/1 -> MATLAB Function1/2(B)
  MATLAB Function1/2(beta) -> β/1
  abc/1 -> MATLAB Function1/1(abc)
  MATLAB Function1/1(alpha) -> α/1
